simulink model "boost_converter_fuzzy"  (R2026a)
settings: Solver=ode15s  StopTime=0.5  MaxStep=1e-4  RelTol=1e-5  AbsTol=1e-7
undefined symbols (not defined in the file or in its folder): C, L, rL, Rload, Vin, Vref
settings Model: Creator=akash  LastModifiedBy=akash

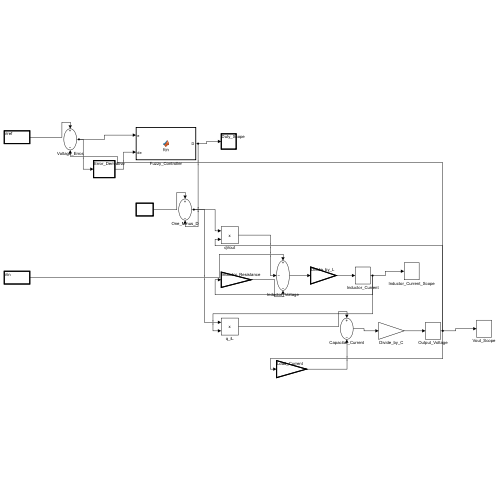
[thumbnail: Simulink's stored preview of the top-level diagram]
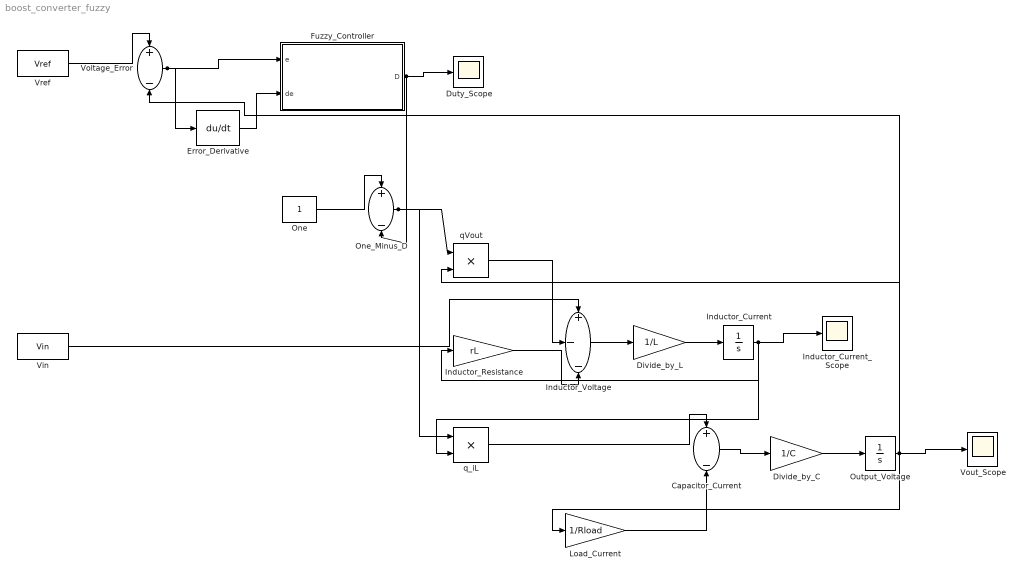
== system boost_converter_fuzzy ==
  Capacitor_Current : Sum  Inputs=+-
  Divide_by_C : Gain  Gain=1/C
  Divide_by_L : Gain  Gain=1/L
  Duty_Scope : Scope
  Error_Derivative : Derivative
  Fuzzy_Controller : MATLAB Function  TreatAsAtomicUnit=on
  Inductor_Current : Integrator
  Inductor_Current_Scope : Scope
  Inductor_Resistance : Gain  Gain=rL
  Inductor_Voltage : Sum  Inputs=+--
  Load_Current : Gain  Gain=1/Rload
  One : Constant
  One_Minus_D : Sum  Inputs=+-
  Output_Voltage : Integrator
  Vin : Constant  Value=Vin
  Voltage_Error : Sum  Inputs=+-
  Vout_Scope : Scope
  Vref : Constant  Value=Vref
  qVout : Product
  q_iL : Product
  wires:
  Vref/1 -> Voltage_Error/1
  Voltage_Error/1 -> Fuzzy_Controller/1(e), Error_Derivative/1
  Error_Derivative/1 -> Fuzzy_Controller/2(de)
  Fuzzy_Controller/1(D) -> One_Minus_D/2, Duty_Scope/1
  One/1 -> One_Minus_D/1
  Vin/1 -> Inductor_Voltage/1
  One_Minus_D/1 -> qVout/1, q_iL/1
  Output_Voltage/1 -> qVout/2, Load_Current/1, Vout_Scope/1, Voltage_Error/2
  qVout/1 -> Inductor_Voltage/2
  Inductor_Current/1 -> Inductor_Resistance/1, Inductor_Current_Scope/1, q_iL/2
  Inductor_Resistance/1 -> Inductor_Voltage/3
  Inductor_Voltage/1 -> Divide_by_L/1
  Divide_by_L/1 -> Inductor_Current/1
  q_iL/1 -> Capacitor_Current/1
  Load_Current/1 -> Capacitor_Current/2
  Capacitor_Current/1 -> Divide_by_C/1
  Divide_by_C/1 -> Output_Voltage/1

== matlab function boost_converter_fuzzy/Fuzzy_Controller ==
  data: e input; D output; de input
function D = fuzzy_controller(e,de)
%#codegen
% Normalized inputs
en = min(max(e/40,-1),1);
dn = min(max(de/200,-1),1);
% Seven membership-function centers
c = [-1,-2/3,-1/3,0,1/3,2/3,1];
muE = zeros(1,7);
muD = zeros(1,7);
for k=1:7
    muE(k) = max(0,1-abs(en-c(k))/(1/3));
    muD(k) = max(0,1-abs(dn-c(k))/(1/3));
end
% Include the endpoint membership sets
if en <= -1, muE(1)=1; end
if en >= 1,  muE(7)=1; end
if dn <= -1, muD(1)=1; end
if dn >= 1,  muD(7)=1; end
% Sugeno singletons: duty corrections
out = [-0.25,-0.17,-0.0833,0,0.0833,0.17,0.25];
num = 0;
den = 0;
for i=1:7
    for j=1:7
        % Error raises duty; derivative provides damping
        idx = round(4 + (i-4) + 0.5*(j-4));
        idx = min(max(idx,1),7);
        w = muE(i)*muD(j);
        num = num + w*out(idx);
        den = den + w;
    end
end
if den > 1e-9
    correction = num/den;
else
    correction = 0;
end
D = min(max(0.5 + correction,0.05),0.90);
end
